simulink model "FSI08"  (R2024b)
settings: Solver=FixedStepAuto  StartTime=0.0  StopTime=t_stop  FixedStep=Ts  RelTol=1e-3
values from neighbouring files (symbols this model uses):
  b = 350    [FSI03WS.m]    (also in FSI04WS.m = 5; FSI08WS.m = 1.25663706144; FSI09WS.m = 3.14159265359)
  F = 1    [FSI08WS.m]    (also in FSI09WS.m = 10)
  f = chirp_end:(chirp_start/(length(t)-1)):chirp_start    [FSI04WS.m]    (also in FSI08WS.m = 5; FSI09WS.m = 5)
  k = 50000    [FSI04WS.m]    (also in FSI08WS.m = 986.960440109; FSI09WS.m = 15791.3670417; FSI10WS.m = 1480)
  m = 70    [FSI03WS.m]    (also in FSI04WS.m = 2; FSI08WS.m = 1; FSI09WS.m = 4; FSI10WS.m = 2)
  swich = -1    [FSI08WS.m]    (also in FSI09WS.m; FSI10WS.m)
  t_stop = 500    [FSI04WS.m]    (also in FSI07WS.m = 1; FSI08WS.m = 100; FSI09WS.m = 600; FSI10WS.m = 1)
  v0 = 25    [FSI01WS.m]    (also in FSI08WS.m = 0; FSI09WS.m = 0)
  x0 = 1    [FSI04WS.m]    (also in FSI08WS.m = 0; FSI09WS.m = 0)
libraries: simulink x1
settings Model: Creator=fmiro  LastModifiedBy=fmiro

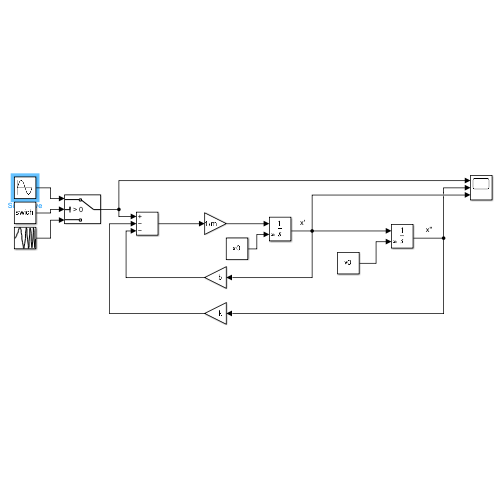
[thumbnail: Simulink's stored preview of the top-level diagram]
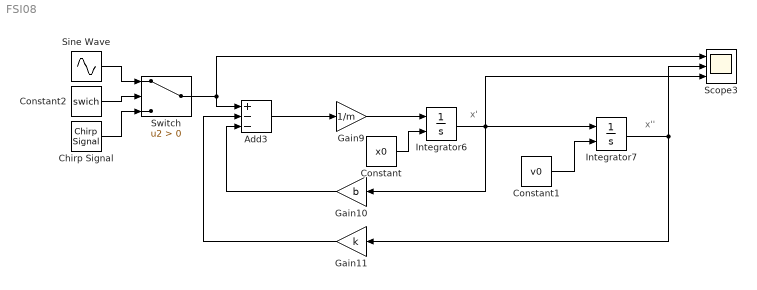
== system FSI08 ==
  note: x''
  note: x'
  Add3 : Sum  Inputs=+--
  Chirp Signal : simulink/Sources/Chirp Signal  f1=0  T=t_stop  f2=20
  Constant : Constant  Value=x0
  Constant1 : Constant  Value=v0
  Constant2 : Constant  Value=swich
  Gain10 : Gain  Gain=b
  Gain11 : Gain  Gain=k
  Gain9 : Gain  Gain=1/m
  Integrator6 : Integrator  InitialConditionSource=external
  Integrator7 : Integrator  InitialConditionSource=external
  Scope3 : Scope  NumInputPorts=3
  Sine Wave : Sin  Amplitude=F  Frequency=2*pi*f  SampleTime=0
  Switch : Switch  Criteria=u2 > Threshold  SaturateOnIntegerOverflow=off  InputSameDT=off
  wires:
  Gain9/1 -> Integrator6/1
  Gain11/1 -> Add3/2
  Integrator6/1 -> Scope3/3, Integrator7/1, Gain10/1
  Add3/1 -> Gain9/1
  Integrator7/1 -> Scope3/2, Gain11/1
  Gain10/1 -> Add3/3
  Constant/1 -> Integrator6/2
  Constant1/1 -> Integrator7/2
  Sine Wave/1 -> Switch/1
  Chirp Signal/1 -> Switch/3
  Switch/1 -> Scope3/1, Add3/1
  Constant2/1 -> Switch/2
